simulink model "grid_afe_n"  (R2026a)
settings: Solver=ode23tb  StopTime=simlength  FixedStep=tc  MaxStep=glb_time.tc
values from neighbouring files (symbols this model uses):
  afe_ctrl = ctrl_afe_setup(glb_time.ts_afe, grid_emu.omega_grid_nom)    [init_model.m]
  afe_pwm_phase_shift_mod1 = 0    [init_model.m]
  afe_pwm_phase_shift_mod2 = 0    [init_model.m]
  afe_pwm_phase_shift_mod3 = 0    [init_model.m]
  afe_pwm_phase_shift_mod4 = 0    [init_model.m]
  filters = setup_global_filters(glb_time.ts_afe, glb_time.ts_inv, glb_time.ts_dab, glb_time.tc)    [init_model.m]
  frt_data = frt_settings(test_index, test_subindex, asymmetric_error_type,      enable_frt_1, enable_frt_2, start_time_LVRT, deepPOSxi, deepPOSeta, deepNEGxi, deepNEGeta)    [init_model.m]
  glb_time = timing_setup(fpwm_afe, trgo_afe, fpwm_inv, trgo_inv, fpwm_single_phase_inv, trgo_single_phase_inv, fpwm_dab, trgo_dab,      fpwm_psfbc, trgo_psfbc, fpwm_isop_rail, trgo_isop_rail, fpwm_cllc, trgo_cllc, t_measure, tc_factor, tc_decimation, delay_pwm, dead_time_afe,      dead_time_inv, dead_time_single_phase_inv, dead_time_dab, dead_time_psfbc, dead_time_isop_rail, dead_time_cllc)    [init_model.m]
  grid_emu = grid_three_phase_emulator('Dyn11', delta_star, grid_nominal_power, application_voltage, us1, us2, fgrid,                  eq_grid_inductance, eq_grid_resistance, eta, ucc, i1m, p_iron, n1, n2, core_area, core_length, mur,                  up_xi_pu_ref, up_eta_pu_ref, un_xi_pu_ref, un_eta_pu_ref)    [init_model.m]
  i_react_pos_ref_2 = -ixi_ref_mod1*tan(acos(0.95))    [init_model.m]
  i_react_pos_ref_3 = ixi_ref_mod1*tan(acos(0.95))    [init_model.m]
  ixi_ref_mod1 = -0.85    [init_model.m]
  ixi_ref_mod2 = -0.85    [init_model.m]
  ixi_ref_mod3 = -0.85    [init_model.m]
  ixi_ref_mod4 = -0.85    [init_model.m]
  ki_align = 18    [init_model.m]
  kp_align = 0.25    [init_model.m]
  lim_down_align = -0.05    [init_model.m]
  lim_up_align = 0.05    [init_model.m]
  mavarage_filter_frequency_base_order = 2    [init_model.m]
  time_gain_afe_module_1 = 1.0002    [init_model.m]
  time_gain_afe_module_2 = 1.0015    [init_model.m]
  time_gain_afe_module_3 = 0.9988    [init_model.m]
  time_gain_afe_module_4 = 1.0020    (= 1.002)    [init_model.m]
  time_i_react_pos_ref_1 = start_time_LVRT + error_length + 0.335    [init_model.m]
  time_i_react_pos_ref_2 = time_i_react_pos_ref_1 + 0.5    (= 0.5)    [init_model.m]
  u_cm_comp_mod1 = 0    [init_model.m]
  u_cm_comp_mod2 = -1    [init_model.m]
  u_cm_comp_mod3 = -1    [init_model.m]
  u_cm_comp_mod4 = -1    [init_model.m]
undefined symbols (not defined in the file or in its folder): hwdata, magnitude
libraries: fl_lib x113, nesl_utility x75, moving_average_filter x40, moving_average_filter_cc x32, sl_discontinuities x12, linear_double_integrator_observer_ccaller x8, discrete_time_low_pass_filter x4, threephase_inductor_lib x4, dclink_for_two_levels x4, three_phase_pwm_modulator x4, three_phase_inverter_ideal_switch_based_model x4, three_phase_inverter_igbt_advanced_thermal_model x4
(part 4 of 19)

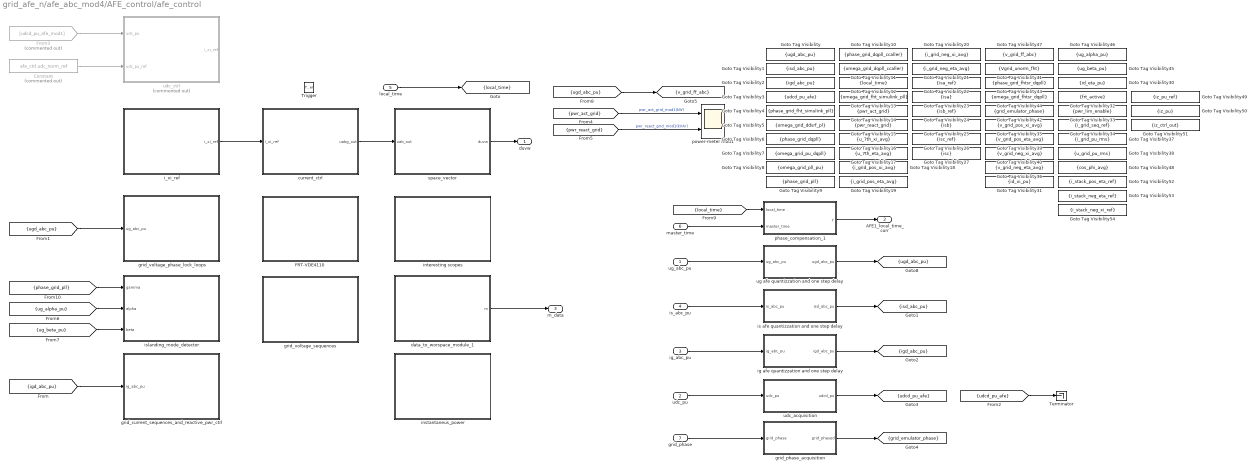
== system grid_afe_n/afe_abc_mod4/AFE_control/afe_control ==
  ug_abc_pu : Inport
  udc_pu : Inport  Port=2
  ig_abc_pu : Inport  Port=3
  is_abc_pu : Inport  Port=4
  local_time : Inport  Port=5
  master_time : Inport  Port=6
  grid_phase : Inport  Port=7
  Trigger : TriggerPort  VariantControl=(inherit)  PortDimensions=1
  Constant : Constant  Commented=on  Value=afe_ctrl.udc_norm_ref
  FRT-VDE4110 : Subsystem
  From3 : From  Commented=on  GotoTag=udcd_pu_afe_mod1  TagVisibility=scoped
  Goto Tag Visibility : GotoTagVisibility  GotoTag=ugd_abc_pu
  Goto Tag Visibility1 : GotoTagVisibility  GotoTag=isd_abc_pu
  Goto Tag Visibility10 : GotoTagVisibility  GotoTag=phase_grid_dqpll_ccaller
  Goto Tag Visibility11 : GotoTagVisibility  GotoTag=omega_grid_dqpll_ccaller
  Goto Tag Visibility12 : GotoTagVisibility  GotoTag=local_time
  Goto Tag Visibility13 : GotoTagVisibility  GotoTag=omega_grid_fht_simulink_pll
  Goto Tag Visibility14 : GotoTagVisibility  GotoTag=pwr_act_grid
  Goto Tag Visibility15 : GotoTagVisibility  GotoTag=pwr_react_grid
  Goto Tag Visibility16 : GotoTagVisibility  GotoTag=u_7th_xi_avg
  Goto Tag Visibility17 : GotoTagVisibility  GotoTag=u_7th_eta_avg
  Goto Tag Visibility18 : GotoTagVisibility  GotoTag=i_grid_pos_xi_avg
  Goto Tag Visibility19 : GotoTagVisibility  GotoTag=i_grid_pos_eta_avg
  Goto Tag Visibility2 : GotoTagVisibility  GotoTag=igd_abc_pu
  Goto Tag Visibility20 : GotoTagVisibility  GotoTag=i_grid_neg_xi_avg
  Goto Tag Visibility21 : GotoTagVisibility  GotoTag=i_grid_neg_eta_avg
  Goto Tag Visibility22 : GotoTagVisibility  GotoTag=isa_ref
  Goto Tag Visibility23 : GotoTagVisibility  GotoTag=isa
  Goto Tag Visibility24 : GotoTagVisibility  GotoTag=isb_ref
  Goto Tag Visibility25 : GotoTagVisibility  GotoTag=isb
  Goto Tag Visibility26 : GotoTagVisibility  GotoTag=isc_ref
  Goto Tag Visibility27 : GotoTagVisibility  GotoTag=isc
  Goto Tag Visibility3 : GotoTagVisibility  GotoTag=udcd_pu_afe
  Goto Tag Visibility30 : GotoTagVisibility  GotoTag=id_eta_pu
  Goto Tag Visibility31 : GotoTagVisibility  GotoTag=id_xi_pu
  Goto Tag Visibility32 : GotoTagVisibility  GotoTag=frt_active
  Goto Tag Visibility33 : GotoTagVisibility  GotoTag=pwr_lim_enable
  Goto Tag Visibility34 : GotoTagVisibility  GotoTag=i_grid_seq_ref
  Goto Tag Visibility35 : GotoTagVisibility  GotoTag=v_grid_pos_xi_avg
  Goto Tag Visibility36 : GotoTagVisibility  GotoTag=v_grid_neg_eta_avg
  Goto Tag Visibility37 : GotoTagVisibility  GotoTag=i_grid_pu_rms
  Goto Tag Visibility38 : GotoTagVisibility  GotoTag=u_grid_pu_rms
  Goto Tag Visibility39 : GotoTagVisibility  GotoTag=v_grid_pos_eta_avg
  Goto Tag Visibility4 : GotoTagVisibility  GotoTag=phase_grid_fht_simulink_pll
  Goto Tag Visibility40 : GotoTagVisibility  GotoTag=v_grid_neg_xi_avg
  Goto Tag Visibility41 : GotoTagVisibility  GotoTag=Vgrid_unorm_fht
  Goto Tag Visibility42 : GotoTagVisibility  GotoTag=grid_emulator_phase
  Goto Tag Visibility43 : GotoTagVisibility  GotoTag=phase_grid_fhtsr_dqpll
  Goto Tag Visibility44 : GotoTagVisibility  GotoTag=omega_grid_fhtsr_dqpll
  Goto Tag Visibility45 : GotoTagVisibility  GotoTag=ug_beta_pu
  Goto Tag Visibility46 : GotoTagVisibility  GotoTag=ug_alpha_pu
  Goto Tag Visibility47 : GotoTagVisibility  GotoTag=v_grid_ff_abc
  Goto Tag Visibility48 : GotoTagVisibility  GotoTag=cos_phi_avg
  Goto Tag Visibility49 : GotoTagVisibility  GotoTag=iz_pu_ref
  Goto Tag Visibility5 : GotoTagVisibility  GotoTag=omega_grid_ddsrf_pl
  Goto Tag Visibility50 : GotoTagVisibility  GotoTag=iz_pu
  Goto Tag Visibility51 : GotoTagVisibility  GotoTag=iz_ctrl_out
  Goto Tag Visibility52 : GotoTagVisibility  GotoTag=i_stack_pos_eta_ref
  Goto Tag Visibility53 : GotoTagVisibility  GotoTag=i_stack_neg_eta_ref
  Goto Tag Visibility54 : GotoTagVisibility  GotoTag=i_stack_neg_xi_ref
  Goto Tag Visibility6 : GotoTagVisibility  GotoTag=phase_grid_dqpll
  Goto Tag Visibility7 : GotoTagVisibility  GotoTag=omega_grid_pu_dqpll
  Goto Tag Visibility8 : GotoTagVisibility  GotoTag=omega_grid_pll_pu
  Goto Tag Visibility9 : GotoTagVisibility  GotoTag=phase_grid_pll
  Terminator : Terminator
  current_ctrl : Subsystem
  data_to_worspace_module_1 : Subsystem
  grid_current_sequences_and_reactive_pwr_ctrl : Subsystem
  grid_phase_acquisition : Subsystem
  grid_voltage_phase_lock_loops : Subsystem
  grid_voltage_sequences : Subsystem
  i_xi_ref : Subsystem
  ig afe quantizzation and one step delay : Subsystem
  instantaneus_power : Subsystem
  interesting scopes : Subsystem
  is afe quantizzation and one step delay : Subsystem
  islanding_mode_detector : Subsystem
  phase_compensation_1 : Subsystem
  power-meter mod1 : Scope  NumInputPorts=2
      settings: ActiveDisplayYMinimum=-42.728052429484045  ActiveDisplayYMaximum=89.297465339663049  DataLoggingVariableName=ScopeData9
  space_vector : Subsystem
  udc_acquisition : Subsystem
  udc_ctrl : Subsystem  Commented=on
  ug afe quantizzation and one step delay : Subsystem
  duvw : Outport
  AFE1_local_time_corr : Outport  Port=2
  m_data : Outport  Port=3
  tag scope: grid_emulator_phase=scoped, igd_abc_pu=scoped, isd_abc_pu=scoped, local_time=scoped, udcd_pu_afe=scoped, ugd_abc_pu=scoped, v_grid_ff_abc=scoped
  wires:
  data_to_worspace_module_1/1(m) -> m_data/1
  i_xi_ref/1(i_xi_ref) -> current_ctrl/1(i_xi_ref)
  [ugd_abc_pu] -> [v_grid_ff_abc]
  grid_phase_acquisition/1(grid_phased) -> [grid_emulator_phase]
  grid_phase/1 -> grid_phase_acquisition/1(grid_phase)
  [local_time] -> phase_compensation_1/1(local_time)
  phase_compensation_1/1(y) -> AFE1_local_time_corr/1
  master_time/1 -> phase_compensation_1/2(master_time)
  local_time/1 -> [local_time]
  [ug_beta_pu] -> islanding_mode_detector/3(beta)
  ig afe quantizzation and one step delay/1(igd_abc_pu) -> [igd_abc_pu]
  is afe quantizzation and one step delay/1(isd_abc_pu) -> [isd_abc_pu]
  ug afe quantizzation and one step delay/1(ugd_abc_pu) -> [ugd_abc_pu]
  [ug_alpha_pu] -> islanding_mode_detector/2(alpha)
  [phase_grid_pll] -> islanding_mode_detector/1(gamma)
  [pwr_act_grid] -> power-meter mod1/1  "pwr_act_grid_mod1(kW)"
  [pwr_react_grid] -> power-meter mod1/2  "pwr_react_grid_mod1(kVAr)"
  udc_acquisition/1(udcd_pu) -> [udcd_pu_afe]
  udc_pu/1 -> udc_acquisition/1(udc_pu)
  From3/1 -> udc_ctrl/1(udc_pu)
  [igd_abc_pu] -> grid_current_sequences_and_reactive_pwr_ctrl/1(ig_abc_pu)
  [ugd_abc_pu] -> grid_voltage_phase_lock_loops/1(ug_abc_pu)
  ig_abc_pu/1 -> ig afe quantizzation and one step delay/1(ig_abc_pu)
  is_abc_pu/1 -> is afe quantizzation and one step delay/1(is_abc_pu)
  space_vector/1(duvw) -> duvw/1
  current_ctrl/1(uabg_out) -> space_vector/1(uab_out)
  ug_abc_pu/1 -> ug afe quantizzation and one step delay/1(ug_abc_pu)
  Constant/1 -> udc_ctrl/2(udc_pu_ref)
  [udcd_pu_afe] -> Terminator/1

== system grid_afe_n/afe_abc_mod4/LCL_filter/threephase_vi_measures_stack ==
  Bus Creator : BusCreator  Inputs=6
  Current Sensor : fl_lib/Electrical/Electrical Sensors/Current Sensor
  Current Sensor1 : fl_lib/Electrical/Electrical Sensors/Current Sensor
  Current Sensor2 : fl_lib/Electrical/Electrical Sensors/Current Sensor
  Electrical Reference1 : fl_lib/Electrical/Electrical Elements/Electrical Reference
  Gain : Gain  Gain=1/3
  Gain1 : Gain  Gain=1/hwdata.afe.ubez
  Gain2 : Gain  Gain=1/hwdata.afe.ubez
  Gain3 : Gain  Gain=1/hwdata.afe.ubez
  Gain4 : Gain  Gain=1/hwdata.afe.ibez
  Gain5 : Gain  Gain=1/hwdata.afe.ibez
  Gain6 : Gain  Gain=1/hwdata.afe.ibez
  Selector : Selector  InputPortWidth=6  IndexOptions=Index vector (dialog)  Indices=[1 2 3]  OutputSizes=1
  Selector1 : Selector  InputPortWidth=6  IndexOptions=Index vector (dialog)  Indices=[4 5 6]  OutputSizes=1
  Sum : Sum  Inputs=+++
  Terminator : Terminator
  Voltage Sensor : fl_lib/Electrical/Electrical Sensors/Voltage Sensor
  Voltage Sensor1 : fl_lib/Electrical/Electrical Sensors/Voltage Sensor
  Voltage Sensor2 : fl_lib/Electrical/Electrical Sensors/Voltage Sensor
  ia_afe : nesl_utility/PS-Simulink Converter  PhysicalDomain=network_engine_domain  SubClassName=ps_output  LeftPortType=input  RightPortType=output  PseudoPeriodic=off  Frequencies=[]  VectorFormat=1-D array  Unit=A  AffineConversion=off
  ib_afe : nesl_utility/PS-Simulink Converter  PhysicalDomain=network_engine_domain  SubClassName=ps_output  LeftPortType=input  RightPortType=output  PseudoPeriodic=off  Frequencies=[]  VectorFormat=1-D array  Unit=A  AffineConversion=off
  ic_afe : nesl_utility/PS-Simulink Converter  PhysicalDomain=network_engine_domain  SubClassName=ps_output  LeftPortType=input  RightPortType=output  PseudoPeriodic=off  Frequencies=[]  VectorFormat=1-D array  Unit=A  AffineConversion=off
  ua_afe : nesl_utility/PS-Simulink Converter  PhysicalDomain=network_engine_domain  SubClassName=ps_output  LeftPortType=input  RightPortType=output  PseudoPeriodic=off  Frequencies=[]  VectorFormat=1-D array  Unit=V  AffineConversion=off
  ub_afe : nesl_utility/PS-Simulink Converter  PhysicalDomain=network_engine_domain  SubClassName=ps_output  LeftPortType=input  RightPortType=output  PseudoPeriodic=off  Frequencies=[]  VectorFormat=1-D array  Unit=V  AffineConversion=off
  uc_afe : nesl_utility/PS-Simulink Converter  PhysicalDomain=network_engine_domain  SubClassName=ps_output  LeftPortType=input  RightPortType=output  PseudoPeriodic=off  Frequencies=[]  VectorFormat=1-D array  Unit=V  AffineConversion=off
  Ua : PMIOPort  Side=Left
  ua : PMIOPort  Port=2  Side=Right
  Ub : PMIOPort  Port=3  Side=Left
  ub : PMIOPort  Port=4  Side=Right
  Uc : PMIOPort  Port=5  Side=Left
  uc : PMIOPort  Port=6  Side=Right
  tag scope: is_abc_pu_mod4=global, iz_afe_pu_mod4=global, vs_abc_pu_mod4=global
  wires:
  Gain5/1 -> Sum/3, Bus Creator/6  "ic_afe_pu"
  Gain4/1 -> Bus Creator/5, Sum/2  "ib_afe_pu"
  Gain6/1 -> Bus Creator/4, Sum/1  "ia_afe_pu"
  Gain3/1 -> Bus Creator/3  "uc_afe_pu"
  Gain2/1 -> Bus Creator/2  "ub_afe_pu"
  Gain1/1 -> Bus Creator/1  "ua_afe_pu"
  Gain/1 -> [iz_afe_pu_mod4]
  Sum/1 -> Gain/1
  Selector1/1 -> [is_abc_pu_mod4]
  uc_afe/1 -> Gain3/1  "uc_afe"
  ub_afe/1 -> Gain2/1  "ub_afe"
  ua_afe/1 -> Gain1/1  "ua_afe"
  ic_afe/1 -> Gain5/1  "ic_afe"
  ia_afe/1 -> Gain6/1  "ia_afe"
  ib_afe/1 -> Gain4/1  "ib_afe"
  Selector/1 -> [vs_abc_pu_mod4]
  Bus Creator/1 -> Selector1/1, Selector/1  "vi_data"
  [vs_abc_pu_mod4] -> Terminator/1
  connections:
  Current Sensor2/RConn2 -- uc/RConn1
  ic_afe/LConn1 -- Current Sensor2/RConn1
  ia_afe/LConn1 -- Current Sensor/RConn1
  ib_afe/LConn1 -- Current Sensor1/RConn1
  Voltage Sensor2/RConn1 -- uc_afe/LConn1
  Current Sensor1/RConn2 -- ub/RConn1
  Voltage Sensor/LConn1 -- Ua/RConn1 -- Current Sensor/LConn1
  Current Sensor2/LConn1 -- Uc/RConn1 -- Voltage Sensor2/LConn1
  Voltage Sensor1/RConn1 -- ub_afe/LConn1
  Current Sensor/RConn2 -- ua/RConn1
  Voltage Sensor/RConn1 -- ua_afe/LConn1
  Voltage Sensor1/RConn2 -- Voltage Sensor2/RConn2 -- Voltage Sensor/RConn2 -- Electrical Reference1/LConn1
  Voltage Sensor1/LConn1 -- Ub/RConn1 -- Current Sensor1/LConn1

== system grid_afe_n/afe_abc_mod4/LCL_filter/threephase_vi_measures_stack1 ==
  Bus Creator : BusCreator  Inputs=6
  Current Sensor : fl_lib/Electrical/Electrical Sensors/Current Sensor
  Current Sensor1 : fl_lib/Electrical/Electrical Sensors/Current Sensor
  Current Sensor2 : fl_lib/Electrical/Electrical Sensors/Current Sensor
  Electrical Reference1 : fl_lib/Electrical/Electrical Elements/Electrical Reference
  Gain1 : Gain  Gain=1/hwdata.afe.ubez
  Gain2 : Gain  Gain=1/hwdata.afe.ubez
  Gain3 : Gain  Gain=1/hwdata.afe.ubez
  Gain4 : Gain  Gain=1/hwdata.afe.ibez
  Gain5 : Gain  Gain=1/hwdata.afe.ibez
  Gain6 : Gain  Gain=1/hwdata.afe.ibez
  Selector : Selector  InputPortWidth=6  IndexOptions=Index vector (dialog)  Indices=[1 2 3]  OutputSizes=1
  Selector1 : Selector  InputPortWidth=6  IndexOptions=Index vector (dialog)  Indices=[4 5 6]  OutputSizes=1
  Voltage Sensor : fl_lib/Electrical/Electrical Sensors/Voltage Sensor
  Voltage Sensor1 : fl_lib/Electrical/Electrical Sensors/Voltage Sensor
  Voltage Sensor2 : fl_lib/Electrical/Electrical Sensors/Voltage Sensor
  ia_grid : nesl_utility/PS-Simulink Converter  PhysicalDomain=network_engine_domain  SubClassName=ps_output  LeftPortType=input  RightPortType=output  PseudoPeriodic=off  Frequencies=[]  VectorFormat=1-D array  Unit=A  AffineConversion=off
  ib_grid : nesl_utility/PS-Simulink Converter  PhysicalDomain=network_engine_domain  SubClassName=ps_output  LeftPortType=input  RightPortType=output  PseudoPeriodic=off  Frequencies=[]  VectorFormat=1-D array  Unit=A  AffineConversion=off
  ic_grid : nesl_utility/PS-Simulink Converter  PhysicalDomain=network_engine_domain  SubClassName=ps_output  LeftPortType=input  RightPortType=output  PseudoPeriodic=off  Frequencies=[]  VectorFormat=1-D array  Unit=A  AffineConversion=off
  ua_grid : nesl_utility/PS-Simulink Converter  PhysicalDomain=network_engine_domain  SubClassName=ps_output  LeftPortType=input  RightPortType=output  PseudoPeriodic=off  Frequencies=[]  VectorFormat=1-D array  Unit=V  AffineConversion=off
  ub_grid : nesl_utility/PS-Simulink Converter  PhysicalDomain=network_engine_domain  SubClassName=ps_output  LeftPortType=input  RightPortType=output  PseudoPeriodic=off  Frequencies=[]  VectorFormat=1-D array  Unit=V  AffineConversion=off
  uc_grid : nesl_utility/PS-Simulink Converter  PhysicalDomain=network_engine_domain  SubClassName=ps_output  LeftPortType=input  RightPortType=output  PseudoPeriodic=off  Frequencies=[]  VectorFormat=1-D array  Unit=V  AffineConversion=off
  Ua : PMIOPort  Side=Left
  ua : PMIOPort  Port=2  Side=Right
  Ub : PMIOPort  Port=3  Side=Left
  ub : PMIOPort  Port=4  Side=Right
  Uc : PMIOPort  Port=5  Side=Left
  uc : PMIOPort  Port=6  Side=Right
  tag scope: ig_abc_pu_mod4=global, ug_abc_pu_mod4=global
  wires:
  Gain5/1 -> Bus Creator/6  "ic_grid_pu"
  Gain4/1 -> Bus Creator/5  "ib_grid_pu"
  Gain6/1 -> Bus Creator/4  "ia_grid_pu"
  Gain3/1 -> Bus Creator/3  "uc_grid_pu"
  Gain2/1 -> Bus Creator/2  "ub_grid_pu"
  Gain1/1 -> Bus Creator/1  "ua_grid_pu"
  Bus Creator/1 -> Selector/1, Selector1/1  "vi_data"
  Selector/1 -> [ug_abc_pu_mod4]
  ib_grid/1 -> Gain4/1
  ia_grid/1 -> Gain6/1
  ic_grid/1 -> Gain5/1
  ua_grid/1 -> Gain1/1
  ub_grid/1 -> Gain2/1
  uc_grid/1 -> Gain3/1
  Selector1/1 -> [ig_abc_pu_mod4]
  connections:
  Ub/RConn1 -- Current Sensor1/LConn1 -- Voltage Sensor1/LConn1
  Electrical Reference1/LConn1 -- Voltage Sensor/RConn2 -- Voltage Sensor2/RConn2 -- Voltage Sensor1/RConn2
  Voltage Sensor/RConn1 -- ua_grid/LConn1
  Current Sensor/RConn2 -- ua/RConn1
  Voltage Sensor1/RConn1 -- ub_grid/LConn1
  Uc/RConn1 -- Voltage Sensor2/LConn1 -- Current Sensor2/LConn1
  Ua/RConn1 -- Current Sensor/LConn1 -- Voltage Sensor/LConn1
  Current Sensor1/RConn2 -- ub/RConn1
  Voltage Sensor2/RConn1 -- uc_grid/LConn1
  ib_grid/LConn1 -- Current Sensor1/RConn1
  ia_grid/LConn1 -- Current Sensor/RConn1
  ic_grid/LConn1 -- Current Sensor2/RConn1
  Current Sensor2/RConn2 -- uc/RConn1

== system grid_afe_n/afe_abc_mod4/afe/sv_pwm ==
  duties_uvw : Inport
  Bus Selector2 : BusSelector  OutputSignals=du(k),dv(k),dw(k)
  Constant1 : Constant  Value=afe_pwm_phase_shift_mod4
  modulator1 : Subsystem
  td2tc_1 : TransferFcn  Denominator=[glb_time.tc 1]
  td2tc_2 : TransferFcn  Denominator=[glb_time.tc 1]
  td2tc_3 : TransferFcn  Denominator=[glb_time.tc 1]
  gate_cmds : Outport
  wires:
  td2tc_2/1 -> modulator1/2(v)  "dv(t)"
  td2tc_3/1 -> modulator1/3(w)  "dw(t)"
  td2tc_1/1 -> modulator1/1(u)  "du(t)"
  duties_uvw/1 -> Bus Selector2/1
  Bus Selector2/3 -> td2tc_3/1  "<dw(k)>"
  Bus Selector2/2 -> td2tc_2/1  "<dv(k)>"
  Bus Selector2/1 -> td2tc_1/1  "<du(k)>"
  Constant1/1 -> modulator1/4(phase)
  modulator1/1(gate_cmds) -> gate_cmds/1

== system grid_afe_n/afe_abc_mod4/afe/three_phase_inverter_ideal_switch_based_model ==
  gate_commands : Inport
  Terminator : Terminator
  three_phase_inverter_ideal_switch_based_model : three_phase_inverter_ideal_switch_based_model/three phase inverter ideal switch based model  Ron_ideal_switch=ideal_switch.Rds_on  Vth=ideal_switch.Vth  Vgamma=ideal_switch.Vdon_diode  Rdon_diode=ideal_switch.Rdon_diode  Csnubber=ideal_switch.Csnubber  Rsnubber=ideal_switch.Rsnubber
  udc(+) : PMIOPort  Side=Left
  u : PMIOPort  Port=2  Side=Right
  v : PMIOPort  Port=3  Side=Right
  udc(-) : PMIOPort  Port=4  Side=Left
  w : PMIOPort  Port=5  Side=Right
  wires:
  gate_commands/1 -> three_phase_inverter_ideal_switch_based_model/1
  three_phase_inverter_ideal_switch_based_model/1 -> Terminator/1
  connections:
  three_phase_inverter_ideal_switch_based_model/RConn3 -- w/RConn1
  three_phase_inverter_ideal_switch_based_model/RConn1 -- u/RConn1
  three_phase_inverter_ideal_switch_based_model/LConn2 -- udc(-)/RConn1
  three_phase_inverter_ideal_switch_based_model/LConn1 -- udc(+)/RConn1
  three_phase_inverter_ideal_switch_based_model/RConn2 -- v/RConn1

== system grid_afe_n/afe_abc_mod4/afe/three_phase_inverter_igbt_based_with_thermal_model ==
  gate_commands : Inport
  three_phase_inverter_igbt_adv_thermal_model : three_phase_inverter_igbt_advanced_thermal_model/three_phase_inverter_igbt_adv_thermal_model  mass_heatsink_m=weigth  specific_heat_m=cp_al  rth_switch_HA_m=Rth_switch_HA  rth_switch_JH_m=igbt.afe.Rth_switch_JH  rth_diode_HA_m=igbt.afe.Rth_diode_CH  rth_diode_JH_m=igbt.afe.Rth_diode_JH  Rce_on_m=igbt.afe.Rce_on  Vce_sat_m=igbt.afe.Vce_sat  Vth_m=igbt.afe.Vth  Eon_m=igbt.afe.Eon  Eoff_m=igbt.afe.Eoff  Erec_m=igbt.afe.Erec  Irr_m=igbt.afe.Irr  Voff_sw_loss_m=igbt.afe.Voff_sw_losses  Ion_sw_loss_m=igbt.afe.Ion_sw_losses  Vdon_diode_m=igbt.afe.Vdon_diode  Rdon_diode_m=igbt.afe.Rdon_diode  Csnubber_m=igbt.afe.Csnubber  Rsnubber_m=igbt.afe.Rsnubber  JunctionTermalMass_m=igbt.afe.JunctionTermalMass  Tambient_m=Tambient  DThs_init_m=DThs_init  Lstray_module_m=igbt.afe.Lstray_module  Cies_m=igbt.afe.Cies  tc_m=glb_time.tc
  u : PMIOPort  Side=Right
  udc(+) : PMIOPort  Port=2  Side=Left
  v : PMIOPort  Port=3  Side=Right
  udc(-) : PMIOPort  Port=4  Side=Left
  w : PMIOPort  Port=5  Side=Right
  wires:
  gate_commands/1 -> three_phase_inverter_igbt_adv_thermal_model/1
  connections:
  three_phase_inverter_igbt_adv_thermal_model/RConn3 -- w/RConn1
  three_phase_inverter_igbt_adv_thermal_model/RConn2 -- v/RConn1
  three_phase_inverter_igbt_adv_thermal_model/LConn1 -- udc(+)/RConn1
  three_phase_inverter_igbt_adv_thermal_model/LConn2 -- udc(-)/RConn1
  three_phase_inverter_igbt_adv_thermal_model/RConn1 -- u/RConn1

== system grid_afe_n/afe_abc_mod4/afe/three_phase_inverter_mosfet_based_with_thermal_model ==
  gate_commands : Inport
  three phase inverter mosfet based with thermal model : three_phase_inverter_mosfet_based_with_thermal_model/three phase inverter mosfet based with thermal model  mass_heatsink_m=0.2  specific_heat_m=880  rth_mosfet_HA_m=0.02  rth_mosfet_JH_m=0.075  Rds_on_m=0.00185  Vth_m=7.5  Eon_m=0.077  Eoff_m=0.108  Voff_sw_loss_m=1300  Ion_sw_loss_m=1000  Vdon_diode_m=4  Rdon_diode_m=0.00185  JunctionTermalMass_m=2  Tambient_m=40  DThs_init_m=0
  u : PMIOPort  Side=Right
  udc(+) : PMIOPort  Port=2  Side=Left
  v : PMIOPort  Port=3  Side=Right
  udc(-) : PMIOPort  Port=4  Side=Left
  w : PMIOPort  Port=5  Side=Right
  wires:
  gate_commands/1 -> three phase inverter mosfet based with thermal model/1
  connections:
  three phase inverter mosfet based with thermal model/RConn1 -- u/RConn1
  three phase inverter mosfet based with thermal model/LConn2 -- udc(-)/RConn1
  three phase inverter mosfet based with thermal model/LConn1 -- udc(+)/RConn1
  three phase inverter mosfet based with thermal model/RConn2 -- v/RConn1
  three phase inverter mosfet based with thermal model/RConn3 -- w/RConn1

== system grid_afe_n/grid/grid_emulator/3ph_Dyg ==
  Electrical Reference1 : fl_lib/Electrical/Electrical Elements/Electrical Reference
  ph1 : single_phase_transformer_lib/single phase transformer  Lm=grid_emu.trafo.Lm1 H  n1=grid_emu.trafo.n1  n2=grid_emu.trafo.n2  Rd1=grid_emu.trafo.Rd1 Ohm  Rd2=grid_emu.trafo.Rd2 Ohm  Ld1=grid_emu.trafo.Ld1 H  Ld2=grid_emu.trafo.Ld2 H  Rfe=grid_emu.trafo.Rfe1 Ohm  phi_specify=off  phi_priority=None  phi=0 V*s  phi_nominal_specify=off  phi_nominal_value=1  phi_nominal_unit=V*s  i1_specify=off  i1_priority=None  i1=0 A  i1_nominal_specify=off  i1_nominal_value=1  i1_nominal_unit=A  i2_specify=off  i2_priority=None  i2=0 A  i2_nominal_specify=off  i2_nominal_value=1  i2_nominal_unit=A  ife_specify=off  ife_priority=None  ife=0 A  ife_nominal_specify=off  ife_nominal_value=1  ife_nominal_unit=A  u1_specify=off  u1_priority=None  u1=0 V  u1_nominal_specify=off  u1_nominal_value=1  u1_nominal_unit=V  u2_specify=off  u2_priority=None  u2=0 V  u2_nominal_specify=off  u2_nominal_value=1  u2_nominal_unit=V
  ph2 : single_phase_transformer_lib/single phase transformer  Lm=grid_emu.trafo.Lm1 H  n1=grid_emu.trafo.n1  n2=grid_emu.trafo.n2  Rd1=grid_emu.trafo.Rd1 Ohm  Rd2=grid_emu.trafo.Rd2 Ohm  Ld1=grid_emu.trafo.Ld1 H  Ld2=grid_emu.trafo.Ld2 H  Rfe=grid_emu.trafo.Rfe1 Ohm  phi_specify=off  phi_priority=None  phi=0 V*s  phi_nominal_specify=off  phi_nominal_value=1  phi_nominal_unit=V*s  i1_specify=off  i1_priority=None  i1=0 A  i1_nominal_specify=off  i1_nominal_value=1  i1_nominal_unit=A  i2_specify=off  i2_priority=None  i2=0 A  i2_nominal_specify=off  i2_nominal_value=1  i2_nominal_unit=A  ife_specify=off  ife_priority=None  ife=0 A  ife_nominal_specify=off  ife_nominal_value=1  ife_nominal_unit=A  u1_specify=off  u1_priority=None  u1=0 V  u1_nominal_specify=off  u1_nominal_value=1  u1_nominal_unit=V  u2_specify=off  u2_priority=None  u2=0 V  u2_nominal_specify=off  u2_nominal_value=1  u2_nominal_unit=V
  ph3 : single_phase_transformer_lib/single phase transformer  Lm=grid_emu.trafo.Lm1 H  n1=grid_emu.trafo.n1  n2=grid_emu.trafo.n2  Rd1=grid_emu.trafo.Rd1 Ohm  Rd2=grid_emu.trafo.Rd2 Ohm  Ld1=grid_emu.trafo.Ld1 H  Ld2=grid_emu.trafo.Ld2 H  Rfe=grid_emu.trafo.Rfe1 Ohm  phi_specify=off  phi_priority=None  phi=0 V*s  phi_nominal_specify=off  phi_nominal_value=1  phi_nominal_unit=V*s  i1_specify=off  i1_priority=None  i1=0 A  i1_nominal_specify=off  i1_nominal_value=1  i1_nominal_unit=A  i2_specify=off  i2_priority=None  i2=0 A  i2_nominal_specify=off  i2_nominal_value=1  i2_nominal_unit=A  ife_specify=off  ife_priority=None  ife=0 A  ife_nominal_specify=off  ife_nominal_value=1  ife_nominal_unit=A  u1_specify=off  u1_priority=None  u1=0 V  u1_nominal_specify=off  u1_nominal_value=1  u1_nominal_unit=V  u2_specify=off  u2_priority=None  u2=0 V  u2_nominal_specify=off  u2_nominal_value=1  u2_nominal_unit=V
  ua : PMIOPort  Side=Right
  ub : PMIOPort  Port=2  Side=Right
  uc : PMIOPort  Port=3  Side=Right
  Ua : PMIOPort  Port=4  Side=Left
  Ub : PMIOPort  Port=5  Side=Left
  Uc : PMIOPort  Port=6  Side=Left
  connections:
  Electrical Reference1/LConn1 -- ph3/RConn2 -- ph2/RConn2 -- ph1/RConn2
  ph3/RConn1 -- uc/RConn1
  ph1/LConn1 -- ph3/LConn2 -- Ua/RConn1
  ph1/RConn1 -- ua/RConn1
  ph2/RConn1 -- ub/RConn1
  ph1/LConn2 -- ph2/LConn1 -- Ub/RConn1
  Uc/RConn1 -- ph3/LConn1 -- ph2/LConn2

== system grid_afe_n/grid/grid_emulator/threephase_vi_measures ==
  Bus Creator : BusCreator  Inputs=6
  Current Sensor : fl_lib/Electrical/Electrical Sensors/Current Sensor
  Current Sensor1 : fl_lib/Electrical/Electrical Sensors/Current Sensor
  Current Sensor2 : fl_lib/Electrical/Electrical Sensors/Current Sensor
  Electrical Reference1 : fl_lib/Electrical/Electrical Elements/Electrical Reference
  Terminator : Terminator
  Terminator1 : Terminator
  Voltage Sensor : fl_lib/Electrical/Electrical Sensors/Voltage Sensor
  Voltage Sensor1 : fl_lib/Electrical/Electrical Sensors/Voltage Sensor
  Voltage Sensor2 : fl_lib/Electrical/Electrical Sensors/Voltage Sensor
  i : Selector  InputPortWidth=6  IndexOptions=Index vector (dialog)  Indices=[4 5 6]  OutputSizes=1
  ia_grid : nesl_utility/PS-Simulink Converter  PhysicalDomain=network_engine_domain  SubClassName=ps_output  LeftPortType=input  RightPortType=output  PseudoPeriodic=off  Frequencies=[]  VectorFormat=1-D array  Unit=A  AffineConversion=off
  ib_grid : nesl_utility/PS-Simulink Converter  PhysicalDomain=network_engine_domain  SubClassName=ps_output  LeftPortType=input  RightPortType=output  PseudoPeriodic=off  Frequencies=[]  VectorFormat=1-D array  Unit=A  AffineConversion=off
  ic_grid : nesl_utility/PS-Simulink Converter  PhysicalDomain=network_engine_domain  SubClassName=ps_output  LeftPortType=input  RightPortType=output  PseudoPeriodic=off  Frequencies=[]  VectorFormat=1-D array  Unit=A  AffineConversion=off
  u : Selector  InputPortWidth=6  IndexOptions=Index vector (dialog)  Indices=[1 2 3]  OutputSizes=1
  ua_grid : nesl_utility/PS-Simulink Converter  PhysicalDomain=network_engine_domain  SubClassName=ps_output  LeftPortType=input  RightPortType=output  PseudoPeriodic=off  Frequencies=[]  VectorFormat=1-D array  Unit=V  AffineConversion=off
  ub_grid : nesl_utility/PS-Simulink Converter  PhysicalDomain=network_engine_domain  SubClassName=ps_output  LeftPortType=input  RightPortType=output  PseudoPeriodic=off  Frequencies=[]  VectorFormat=1-D array  Unit=V  AffineConversion=off
  uc_grid : nesl_utility/PS-Simulink Converter  PhysicalDomain=network_engine_domain  SubClassName=ps_output  LeftPortType=input  RightPortType=output  PseudoPeriodic=off  Frequencies=[]  VectorFormat=1-D array  Unit=V  AffineConversion=off
  Ua : PMIOPort  Side=Left
  ua : PMIOPort  Port=2  Side=Right
  Ub : PMIOPort  Port=3  Side=Left
  ub : PMIOPort  Port=4  Side=Right
  Uc : PMIOPort  Port=5  Side=Left
  uc : PMIOPort  Port=6  Side=Right
  tag scope: i_abc_line=global, u_abc_line=global
  wires:
  Bus Creator/1 -> i/1, u/1  "vi_data"
  ib_grid/1 -> Bus Creator/5  "ib"
  ia_grid/1 -> Bus Creator/4  "ia"
  ic_grid/1 -> Bus Creator/6  "ic"
  ua_grid/1 -> Bus Creator/1  "ua"
  ub_grid/1 -> Bus Creator/2  "ub"
  uc_grid/1 -> Bus Creator/3  "uc"
  i/1 -> [i_abc_line]
  u/1 -> [u_abc_line]
  [u_abc_line] -> Terminator/1
  [i_abc_line] -> Terminator1/1
  connections:
  Current Sensor1/LConn1 -- Ub/RConn1 -- Voltage Sensor1/LConn1
  Electrical Reference1/LConn1 -- Voltage Sensor/RConn2 -- Voltage Sensor2/RConn2 -- Voltage Sensor1/RConn2
  Voltage Sensor/RConn1 -- ua_grid/LConn1
  Current Sensor/RConn2 -- ua/RConn1
  Voltage Sensor1/RConn1 -- ub_grid/LConn1
  Voltage Sensor2/LConn1 -- Current Sensor2/LConn1 -- Uc/RConn1
  Current Sensor/LConn1 -- Ua/RConn1 -- Voltage Sensor/LConn1
  Current Sensor1/RConn2 -- ub/RConn1
  Voltage Sensor2/RConn1 -- uc_grid/LConn1
  ib_grid/LConn1 -- Current Sensor1/RConn1
  ia_grid/LConn1 -- Current Sensor/RConn1
  ic_grid/LConn1 -- Current Sensor2/RConn1
  Current Sensor2/RConn2 -- uc/RConn1

== system grid_afe_n/afe_abc_mod1/AFE_control/afe_control/FRT-VDE4110 ==
  Constant : Constant  Value=0
  FRT-Detection : Subsystem
  FRT-PosNegReactiveCurrentReferences : Subsystem
  Terminator : Terminator
  Terminator1 : Terminator
  frt_detection_output : Scope  NumInputPorts=3
      settings: ActiveDisplayYMinimum=-0.12499999999999997  ActiveDisplayYMaximum=1.125
  tag scope: frt_active=scoped, pwr_lim_enable=scoped
  wires:
  [v_grid_pos_xi_avg] -> FRT-PosNegReactiveCurrentReferences/1(In1)
  [v_grid_neg_xi_avg] -> FRT-PosNegReactiveCurrentReferences/3(In3)
  [v_grid_neg_eta_avg] -> FRT-PosNegReactiveCurrentReferences/4(In4)
  [v_grid_pos_eta_avg] -> FRT-PosNegReactiveCurrentReferences/2(In2)
  FRT-Detection/4(frt_active) -> frt_detection_output/2, [frt_active]  "frt_active"
  FRT-Detection/5(pwr_lim_enable) -> frt_detection_output/3, [pwr_lim_enable]  "pwr_lim_enable"
  FRT-Detection/2(frt_state) -> frt_detection_output/1  "frt_state"
  Constant/1 -> FRT-Detection/1(red_dyn_enabled)
  FRT-Detection/1(frt_exceeded) -> Terminator/1
  FRT-Detection/3(red_dyn_active) -> Terminator1/1

== system grid_afe_n/afe_abc_mod1/AFE_control/afe_control/current_ctrl ==
  i_xi_ref : Inport
  Demux : Demux  Outputs=3
  current_transformation : Subsystem
  inner_current_ctrl : Subsystem
  xieta2abc : Subsystem
  uabg_out : Outport
  wires:
  Demux/1 -> current_transformation/1(is_a_pu)  "is_a"
  Demux/2 -> current_transformation/2(is_b_pu)  "is_b"
  Demux/3 -> current_transformation/3(is_c_pu)  "is_c"
  [isd_abc_pu] -> Demux/1
  [phase_grid_pll] -> xieta2abc/5(phase)
  xieta2abc/1(i_abc) -> inner_current_ctrl/1(In1)
  [isd_abc_pu] -> inner_current_ctrl/2(is_abc)
  inner_current_ctrl/1(uabg) -> uabg_out/1
  i_xi_ref/1 -> xieta2abc/1(pos_xi)  "i_xi_ref"
  [i_stack_neg_eta_ref] -> xieta2abc/4(neg_eta)
  [i_stack_neg_xi_ref] -> xieta2abc/3(neg_xi)
  [i_stack_pos_eta_ref] -> xieta2abc/2(pos_eta)

== system grid_afe_n/afe_abc_mod1/AFE_control/afe_control/data_to_worspace_module_1 ==
  Bus Creator : BusCreator  Inputs=5
  dq_pll : Subsystem
  inner_current_tracking : Subsystem
  pwr_meter : Subsystem
  sequences_data : Subsystem
  m : Outport
  wires:
  Bus Creator/1 -> m/1
  sequences_data/1(m_seq) -> Bus Creator/1  "sequences_data"
  pwr_meter/1(m_pwr_meter) -> Bus Creator/2  "pwr_meter"
  inner_current_tracking/1(m_inner_current_tracking) -> Bus Creator/3  "m_inner_current_tracking"
  [local_time] -> Bus Creator/5  "local_time"
  dq_pll/1(dqPLLs) -> Bus Creator/4  "dq_pll"

== system grid_afe_n/afe_abc_mod1/AFE_control/afe_control/grid_current_sequences_and_reactive_pwr_ctrl ==
  ig_abc_pu : Inport
  current_sequence_avg : Subsystem
  grid_current_sampling_and_alpha_beta_transformation : Subsystem
  i_alphabeta2xieta : Subsystem
  sequences_current_control : Subsystem
  tag scope: i_grid_neg_eta_avg=scoped, i_grid_neg_xi_avg=scoped, i_grid_pos_eta_avg=scoped, i_grid_pos_xi_avg=scoped
  wires:
  i_alphabeta2xieta/1(xi) -> current_sequence_avg/1(i_grid_pos_xi)
  i_alphabeta2xieta/3(v_grid_neg_xi) -> current_sequence_avg/3(i_grid_neg_xi)
  i_alphabeta2xieta/4(e) -> current_sequence_avg/4(i_grid_neg_eta)
  current_sequence_avg/4(i_grid_neg_eta_avg) -> sequences_current_control/4(i_neg_eta), [i_grid_neg_eta_avg]
  ig_abc_pu/1 -> grid_current_sampling_and_alpha_beta_transformation/1(ig_abc)
  i_alphabeta2xieta/2(v_grid_pos_eta) -> current_sequence_avg/2(i_grid_pos_eta)
  current_sequence_avg/1(i_grid_pos_xi_avg) -> [i_grid_pos_xi_avg], sequences_current_control/1(i_pos_xi)
  current_sequence_avg/2(i_grid_pos_eta_avg) -> [i_grid_pos_eta_avg], sequences_current_control/2(i_pos_eta)
  [phase_grid_pll] -> i_alphabeta2xieta/3(gamma)
  grid_current_sampling_and_alpha_beta_transformation/2(i_grid_beta) -> i_alphabeta2xieta/2(beta)
  grid_current_sampling_and_alpha_beta_transformation/1(i_grid_alpha) -> i_alphabeta2xieta/1(alpha)
  current_sequence_avg/3(i_grid_neg_xi_avg) -> sequences_current_control/3(i_neg_xi), [i_grid_neg_xi_avg]

== system grid_afe_n/afe_abc_mod1/AFE_control/afe_control/grid_phase_acquisition ==
  grid_phase : Inport
  Quantizer : Quantizer  QuantizationInterval=adc_quantization
  Unit Delay : UnitDelay  SampleTime=-1
  Zero-Order Hold : ZeroOrderHold  SampleTime=-1
  grid_phased : Outport
  wires:
  Zero-Order Hold/1 -> Quantizer/1
  Unit Delay/1 -> grid_phased/1
  grid_phase/1 -> Zero-Order Hold/1
  Quantizer/1 -> Unit Delay/1

== system grid_afe_n/afe_abc_mod1/AFE_control/afe_control/grid_voltage_phase_lock_loops ==
  ug_abc_pu : Inport
  Bus Creator : BusCreator  Inputs=5
  Bus Creator1 : BusCreator  Inputs=4
  Bus Creator2 : BusCreator  Inputs=2
  FHT-PLL : Subsystem
  FHT-PLL performance : Scope  NumInputPorts=2
      settings: ActiveDisplayYMinimum=-1.251220703125  ActiveDisplayYMaximum=1.251220703125  DataLoggingVariableName=ScopeData8
  FHT-PLL_simulink : Subsystem
  Variant Source1 : VariantSource  VariantControls={use_dq_pll_mode1 == 1, use_dq_pll_mode2 == 1, use_dq_pll_mode3 == 1, use_dq_pll_mode4 == 1}
  Variant Source2 : VariantSource  VariantControls={use_dq_pll_mode1 == 1, use_dq_pll_mode2 == 1, use_dq_pll_mode3 == 1, use_dq_pll_mode4 == 1}
  dq_pll : Subsystem
  dq_pll_ccaller : Subsystem
  dqpll_ccaler : Scope  NumInputPorts=3
      settings: ActiveDisplayYMinimum=-0.88802937790751446  ActiveDisplayYMaximum=4.5431143753230572  DataLoggingVariableName=ScopeData4
  pll_performances : Scope  NumInputPorts=2
      settings: ActiveDisplayYMinimum=-3.927001953125  ActiveDisplayYMaximum=3.927001953125  DataLoggingVariableName=ScopeData34
  tag scope: omega_grid_dqpll_ccaller=scoped, omega_grid_fht_simulink_pll=scoped, omega_grid_fhtsr_dqpll=scoped, omega_grid_pll_pu=scoped, omega_grid_pu_dqpll=scoped, phase_grid_dqpll=scoped, phase_grid_dqpll_ccaller=scoped, phase_grid_fht_simulink_pll=scoped, phase_grid_fhtsr_dqpll=scoped, phase_grid_pll=scoped
  wires:
  Variant Source1/1 -> [phase_grid_pll]
  FHT-PLL_simulink/1(gamma_grid_fht_pll) -> [phase_grid_fht_simulink_pll]
  FHT-PLL_simulink/2(omega_grid_fht_pll) -> [omega_grid_fht_simulink_pll]
  dq_pll/2(omega_grid_pu_dqpll) -> [omega_grid_pu_dqpll]
  dq_pll/1(phase_grid_dqpll) -> [phase_grid_dqpll]
  dq_pll_ccaller/1(gamma_hat) -> [phase_grid_dqpll_ccaller]
  dq_pll_ccaller/2(omega_pu_hat) -> [omega_grid_dqpll_ccaller]
  [phase_grid_dqpll] -> Variant Source1/1, Bus Creator/1  "phase_grid_dqpll"
  [phase_grid_dqpll_ccaller] -> Bus Creator/2, Variant Source1/2  "phase_grid_dqpll_ccaller"
  [phase_grid_fht_simulink_pll] -> Bus Creator/3, Variant Source1/3  "phase_grid_fht_simulink_pll"
  [omega_grid_pu_dqpll] -> Variant Source2/1, Bus Creator1/1  "omega_grid_pu_dqpll"
  [omega_grid_dqpll_ccaller] -> Variant Source2/2, Bus Creator1/2  "omega_grid_dqpll_ccaller"
  [omega_grid_fht_simulink_pll] -> Variant Source2/3, Bus Creator1/3  "omega_grid_fht_simulink_pll"
  Variant Source2/1 -> [omega_grid_pll_pu]
  dq_pll_ccaller/3(dqpll_uxi) -> dqpll_ccaler/1  "uxi_n"
  dq_pll_ccaller/4(dqpll_ueta) -> dqpll_ccaler/2  "ueta_n"
  dq_pll_ccaller/5(dqpll_state) -> dqpll_ccaler/3  "dqpll_state"
  ug_abc_pu/1 -> FHT-PLL performance/1, dq_pll/1(ug_abc_pu), FHT-PLL_simulink/1(ug_abc_pu), FHT-PLL/1(ug_abc_pu), dq_pll_ccaller/1(ug_abc_pu)
  Bus Creator/1 -> pll_performances/1
  Bus Creator1/1 -> pll_performances/2
  [grid_emulator_phase] -> Bus Creator/4  "grid_emulator_phase"
  FHT-PLL/2(omega_grid_fht_pll) -> [omega_grid_fhtsr_dqpll]
  FHT-PLL/1(gamma_grid_fht_pll) -> [phase_grid_fhtsr_dqpll]
  [phase_grid_fhtsr_dqpll] -> Bus Creator/5  "phase_grid_fht_pll"
  [omega_grid_fhtsr_dqpll] -> Bus Creator1/4  "omega_grid_fht_pll"
  [phase_grid_fhtsr_dqpll] -> Variant Source1/4  "phase_grid_fht_pll"
  [omega_grid_fhtsr_dqpll] -> Variant Source2/4  "omega_grid_fht_pll"
  Bus Creator2/1 -> FHT-PLL performance/2
  [omega_grid_fhtsr_dqpll] -> Bus Creator2/2  "omega_grid_fht_pll"
  [phase_grid_fhtsr_dqpll] -> Bus Creator2/1  "phase_grid_fht_pll"

== system grid_afe_n/afe_abc_mod1/AFE_control/afe_control/grid_voltage_sequences ==
  grid_voltage_sampling_and_alpha_beta_transformation : Subsystem
  v_alphabeta2xieta : Subsystem
  voltage_sequence_avg : Subsystem
  tag scope: ug_alpha_pu=scoped, ug_beta_pu=scoped, v_grid_neg_eta_avg=scoped, v_grid_neg_xi_avg=scoped, v_grid_pos_eta_avg=scoped, v_grid_pos_xi_avg=scoped
  wires:
  v_alphabeta2xieta/4(v_grid_neg_eta) -> voltage_sequence_avg/4(v_grid_neg_eta)  "neg_eta"
  v_alphabeta2xieta/2(eta) -> voltage_sequence_avg/2(v_grid_pos_eta)  "pos_eta"
  [phase_grid_pll] -> v_alphabeta2xieta/3(gamma)
  v_alphabeta2xieta/3(v_grid_neg_xi) -> voltage_sequence_avg/3(v_grid_neg_xi)  "neg_xi"
  voltage_sequence_avg/3(v_grid_neg_xi_avg) -> [v_grid_neg_xi_avg]
  voltage_sequence_avg/2(v_grid_pos_eta_avg) -> [v_grid_pos_eta_avg]
  voltage_sequence_avg/4(v_grid_neg_eta_avg) -> [v_grid_neg_eta_avg]
  grid_voltage_sampling_and_alpha_beta_transformation/2(u_grid_beta) -> [ug_beta_pu], v_alphabeta2xieta/2(beta)
  voltage_sequence_avg/1(v_grid_pos_xi_avg) -> [v_grid_pos_xi_avg]
  v_alphabeta2xieta/1(xi) -> voltage_sequence_avg/1(v_grid_pos_xi)  "pos_xi"
  grid_voltage_sampling_and_alpha_beta_transformation/1(u_grid_alpha) -> [ug_alpha_pu], v_alphabeta2xieta/1(alpha)
  [ugd_abc_pu] -> grid_voltage_sampling_and_alpha_beta_transformation/1(v_abc)

== system grid_afe_n/afe_abc_mod1/AFE_control/afe_control/i_xi_ref ==
  Constant1 : Constant  Value=ixi_ref_mod1
  Constant2 : Constant  Value=0
  Delay : Delay  DelayLength=floor(0.25/glb_time.ts_afe)
  Switch : Switch  Criteria=u2 > Threshold  SaturateOnIntegerOverflow=off  InputSameDT=off
  Switch1 : Switch  Criteria=u2 > Threshold  SaturateOnIntegerOverflow=off  InputSameDT=off
  Variant Source : VariantSource  VariantControls={false, true}
  discrete-time-low-pass-filter : discrete_time_low_pass_filter/discrete-time-low-pass-filter  tau=0.125  ts=glb_time.ts_afe
  i_xi_ref : Outport
  wires:
  Constant1/1 -> Switch/3  "i_xi_ref"
  Constant2/1 -> Switch/1
  [pwr_lim_enable] -> Switch/2
  [pwr_lim_enable] -> Delay/1
  Switch/1 -> discrete-time-low-pass-filter/1, Variant Source/2, Switch1/3
  Delay/1 -> Switch1/2
  discrete-time-low-pass-filter/1 -> Switch1/1
  Switch1/1 -> Variant Source/1
  Variant Source/1 -> i_xi_ref/1

== system grid_afe_n/afe_abc_mod1/AFE_control/afe_control/ig afe quantizzation and one step delay ==
  ig_abc_pu : Inport
  Demux1 : Demux  Outputs=3
  Mux1 : Mux  Inputs=3
  ig afe quantizzation and one step delay : Subsystem
  igd_abc_pu : Outport
  wires:
  Demux1/1 -> ig afe quantizzation and one step delay/1(ig_u_pu)
  Demux1/2 -> ig afe quantizzation and one step delay/2(ig_v_pu)
  ig_abc_pu/1 -> Demux1/1
  Mux1/1 -> igd_abc_pu/1
  Demux1/3 -> ig afe quantizzation and one step delay/3(ig_w_pu)
  ig afe quantizzation and one step delay/2(igd_v_pu) -> Mux1/2
  ig afe quantizzation and one step delay/1(igd_u_pu) -> Mux1/1
  ig afe quantizzation and one step delay/3(igd_w_pu) -> Mux1/3

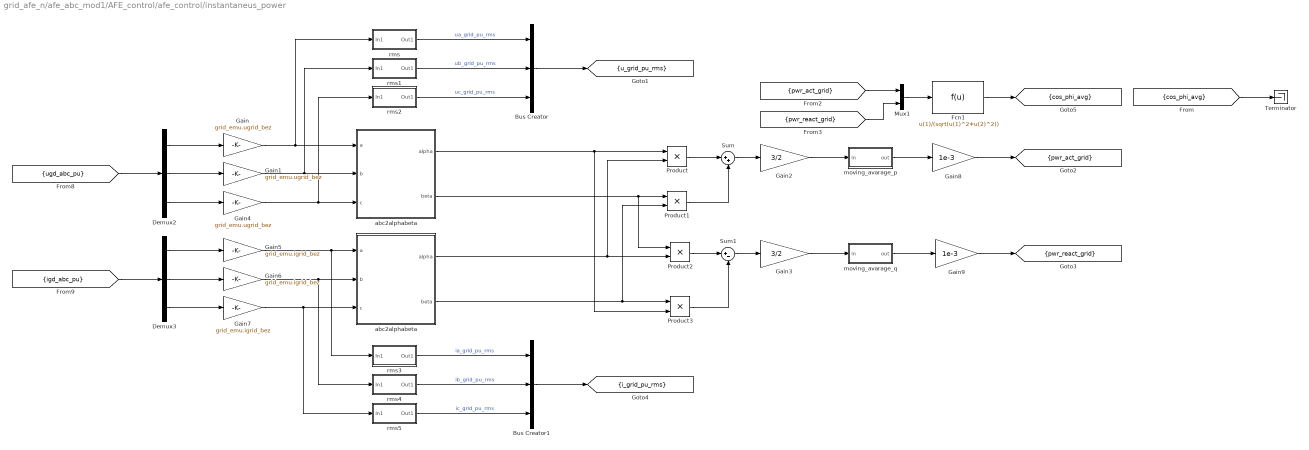
== system grid_afe_n/afe_abc_mod1/AFE_control/afe_control/instantaneus_power ==
  Bus Creator : BusCreator  Inputs=3
  Bus Creator1 : BusCreator  Inputs=3
  Demux2 : Demux  Outputs=3
  Demux3 : Demux  Outputs=3
  Fcn1 : Fcn  Expr=u(1)/(sqrt(u(1)^2+u(2)^2))
  Gain : Gain  Gain=grid_emu.ugrid_bez
  Gain1 : Gain  Gain=grid_emu.ugrid_bez
  Gain2 : Gain  Gain=3/2
  Gain3 : Gain  Gain=3/2
  Gain4 : Gain  Gain=grid_emu.ugrid_bez
  Gain5 : Gain  Gain=grid_emu.igrid_bez
  Gain6 : Gain  Gain=grid_emu.igrid_bez
  Gain7 : Gain  Gain=grid_emu.igrid_bez
  Gain8 : Gain  Gain=1e-3
  Gain9 : Gain  Gain=1e-3
  Mux1 : Mux  Inputs=2
  Product{,1..3} (4 alike) : Product  RndMeth=Zero
  Sum : Sum  Inputs=|++
  Sum1 : Sum  Inputs=|+-
  Terminator : Terminator
  abc2alphabeta : Subsystem
  "abc2alphabeta " : Subsystem
  moving_avarage_p : Subsystem
  moving_avarage_q : Subsystem
  rms : Subsystem
  rms1 : Subsystem
  rms2 : Subsystem
  rms3 : Subsystem
  rms4 : Subsystem
  rms5 : Subsystem
  tag scope: cos_phi_avg=scoped, i_grid_pu_rms=scoped, pwr_act_grid=scoped, pwr_react_grid=scoped, u_grid_pu_rms=scoped
  wires:
  abc2alphabeta/2("beta ") -> Product1/1, Product2/1
  "abc2alphabeta "/2("beta ") -> Product1/2, Product3/1
  abc2alphabeta/1("alpha ") -> Product3/2, Product/1
  "abc2alphabeta "/1("alpha ") -> Product2/2, Product/2
  Product/1 -> Sum/1
  Product1/1 -> Sum/2
  Product2/1 -> Sum1/1
  Product3/1 -> Sum1/2
  Sum1/1 -> Gain3/1
  Sum/1 -> Gain2/1
  Gain2/1 -> moving_avarage_p/1(in)
  Gain3/1 -> moving_avarage_q/1(in)
  [pwr_react_grid] -> Mux1/2
  Mux1/1 -> Fcn1/1
  Fcn1/1 -> [cos_phi_avg]
  [pwr_act_grid] -> Mux1/1
  rms/1(Out1) -> Bus Creator/1  "ua_grid_pu_rms"
  rms2/1(Out1) -> Bus Creator/3  "uc_grid_pu_rms"
  rms1/1(Out1) -> Bus Creator/2  "ub_grid_pu_rms"
  moving_avarage_p/1(out) -> Gain8/1
  moving_avarage_q/1(out) -> Gain9/1
  Demux2/1 -> Gain/1
  Demux2/2 -> Gain1/1
  Demux2/3 -> Gain4/1
  Demux3/1 -> Gain5/1
  Demux3/2 -> Gain6/1
  Demux3/3 -> Gain7/1
  Gain/1 -> rms/1(In1), abc2alphabeta/1(a)
  Gain1/1 -> rms1/1(In1), abc2alphabeta/2(b)
  Gain4/1 -> rms2/1(In1), abc2alphabeta/3(c)
  Gain5/1 -> rms3/1(In1), "abc2alphabeta "/1(a)
  Gain6/1 -> rms4/1(In1), "abc2alphabeta "/2(b)
  Gain7/1 -> rms5/1(In1), "abc2alphabeta "/3(c)
  Gain8/1 -> [pwr_act_grid]
  Gain9/1 -> [pwr_react_grid]
  [ugd_abc_pu] -> Demux2/1
  [igd_abc_pu] -> Demux3/1
  Bus Creator/1 -> [u_grid_pu_rms]
  rms4/1(Out1) -> Bus Creator1/2  "ib_grid_pu_rms"
  rms3/1(Out1) -> Bus Creator1/1  "ia_grid_pu_rms"
  rms5/1(Out1) -> Bus Creator1/3  "ic_grid_pu_rms"
  Bus Creator1/1 -> [i_grid_pu_rms]
  [cos_phi_avg] -> Terminator/1

== system grid_afe_n/afe_abc_mod1/AFE_control/afe_control/interesting scopes ==
  current_sequences_mod1 : Scope  NumInputPorts=4
      settings: ActiveDisplayYMinimum=-0.97178065031766891  ActiveDisplayYMaximum=1.9392475411295891  DataLoggingVariableName=ScopeData2
  i_grid_seq_ref : Scope
      settings: ActiveDisplayYMinimum=-1.1499999999999995  ActiveDisplayYMaximum=0.34999999999999981
  voltage_sequences_mod1 : Scope  NumInputPorts=4
      settings: ActiveDisplayYMinimum=-1.2405151816982258  ActiveDisplayYMaximum=1.2605257614333911
  wires:
  [v_grid_neg_eta_avg] -> voltage_sequences_mod1/4  "u_grid_neg_eta"
  [i_grid_neg_xi_avg] -> current_sequences_mod1/3  "i_grid_neg_xi"
  [v_grid_pos_eta_avg] -> voltage_sequences_mod1/2  "u_grid_pos_eta"
  [v_grid_neg_xi_avg] -> voltage_sequences_mod1/3  "u_grid_neg_xi"
  [i_grid_pos_xi_avg] -> current_sequences_mod1/1  "i_grid_pos_xi"
  [i_grid_neg_eta_avg] -> current_sequences_mod1/4  "i_grid_neg_eta"
  [v_grid_pos_xi_avg] -> voltage_sequences_mod1/1  "u_grid_pos_xi"
  [i_grid_pos_eta_avg] -> current_sequences_mod1/2  "i_grid_pos_eta"
  [i_grid_seq_ref] -> i_grid_seq_ref/1  "i_grid_seq_ref"

== system grid_afe_n/afe_abc_mod1/AFE_control/afe_control/is afe quantizzation and one step delay ==
  is_abc_pu : Inport
  Demux : Demux  Outputs=3
  Mux : Mux  Inputs=3
  is afe quantizzation and one step delay : Subsystem
  isd_abc_pu : Outport
  wires:
  is afe quantizzation and one step delay/2(isd_v_pu) -> Mux/2
  is_abc_pu/1 -> Demux/1
  is afe quantizzation and one step delay/3(isd_w_pu) -> Mux/3
  is afe quantizzation and one step delay/1(isd_u_pu) -> Mux/1
  Demux/1 -> is afe quantizzation and one step delay/1(is_u_pu)
  Mux/1 -> isd_abc_pu/1
  Demux/3 -> is afe quantizzation and one step delay/3(is_w_pu)
  Demux/2 -> is afe quantizzation and one step delay/2(is_v_pu)

== system grid_afe_n/afe_abc_mod1/AFE_control/afe_control/islanding_mode_detector ==
  gamma : Inport
  alpha : Inport  Port=2
  beta : Inport  Port=3
  Gain : Gain  Gain=7
  MATLAB Function : MATLAB Function  TreatAsAtomicUnit=on
  Terminator : Terminator
  Terminator1 : Terminator
  bounder : MATLAB Function  TreatAsAtomicUnit=on
  moving_avarage_1 : Subsystem
  moving_avarage_2 : Subsystem
  seventh_ugrid_component : Scope  NumInputPorts=2
      settings: ActiveDisplayYMinimum=-0.0034745064787606167  ActiveDisplayYMaximum=0.0074022094547510631  DataLoggingVariableName=ScopeData10
  tag scope: u_7th_eta_avg=scoped, u_7th_xi_avg=scoped
  wires:
  gamma/1 -> Gain/1  "gamma_grid"
  MATLAB Function/1(xi) -> moving_avarage_1/1(u)
  bounder/1(y) -> MATLAB Function/3(gamma)
  Gain/1 -> bounder/1(u)
  alpha/1 -> MATLAB Function/1(alpha)  "u_grid_alpha"
  beta/1 -> MATLAB Function/2(beta)  "u_grid_beta"
  MATLAB Function/2(eta) -> moving_avarage_2/1(u)
  moving_avarage_1/1(y) -> [u_7th_xi_avg], seventh_ugrid_component/1  "u_7th_xi"
  moving_avarage_2/1(y) -> [u_7th_eta_avg], seventh_ugrid_component/2  "u_7th_eta"
  [u_7th_xi_avg] -> Terminator/1
  [u_7th_eta_avg] -> Terminator1/1

== system grid_afe_n/afe_abc_mod1/AFE_control/afe_control/phase_compensation_1 ==
  local_time : Inport
  master_time : Inport  Port=2
  Zero-Order Hold : ZeroOrderHold  SampleTime=-1
  Zero-Order Hold1 : ZeroOrderHold  SampleTime=-1
  alignment_eval_afe1 : Subsystem
  y : Outport
  wires:
  local_time/1 -> Zero-Order Hold/1
  master_time/1 -> Zero-Order Hold1/1
  alignment_eval_afe1/1(dp) -> y/1
  Zero-Order Hold/1 -> alignment_eval_afe1/1(local_time)
  Zero-Order Hold1/1 -> alignment_eval_afe1/2(master_time)
